simulink model "Three_Stages"  (R2023a)
settings: Solver=FixedStepDiscrete  StartTime=0.0  StopTime=5000  FixedStep=1  RelTol=1e-3
values from neighbouring files (symbols this model uses):
  fw = zeros(16384, 1, 'uint32')    [test.m]
libraries: hdlsllib x27, simulink x27, etargetslib x1
(part 4 of 5)

== system Three_Stages/Subsystem21/Subsystem17 ==
  rst_n : Inport
  stall : Inport  Port=2
  flush : Inport  Port=3
  s_in : Inport  Port=4
  Constant : Constant  Value=0  OutDataTypeStr=boolean
  Constant1 : Constant  Value=0  OutDataTypeStr=uint32
  Resettable Delay : Delay  DelayLength=1  InitialConditionSource=Input port  ExternalReset=Falling
      settings: InputPortMap=u0,r5,p4
  Switch : Switch  Criteria=u2 ~= 0  OutDataTypeStr=boolean  SaturateOnIntegerOverflow=off  InputSameDT=off
  Switch1 : Switch  Criteria=u2 ~= 0  OutDataTypeStr=boolean  SaturateOnIntegerOverflow=off  InputSameDT=off
  s_out : Outport
  wires:
  Constant1/1 -> Switch1/1
  Switch1/1 -> Resettable Delay/1
  Resettable Delay/1 -> s_out/1, Switch/1
  Constant/1 -> Resettable Delay/3
  flush/1 -> Switch1/2
  rst_n/1 -> Resettable Delay/2
  Switch/1 -> Switch1/3
  stall/1 -> Switch/2
  s_in/1 -> Switch/3

== system Three_Stages/Subsystem21/Subsystem18 ==
  rst_n : Inport
  stall : Inport  Port=2
  flush : Inport  Port=3
  valid_in : Inport  Port=4
  Constant : Constant  Value=0  OutDataTypeStr=boolean
  Constant1 : Constant  Value=0  OutDataTypeStr=uint32
  Resettable Delay : Delay  DelayLength=1  InitialConditionSource=Input port  ExternalReset=Falling
      settings: InputPortMap=u0,r5,p4
  Switch : Switch  Criteria=u2 ~= 0  OutDataTypeStr=boolean  SaturateOnIntegerOverflow=off  InputSameDT=off
  Switch1 : Switch  Criteria=u2 ~= 0  OutDataTypeStr=boolean  SaturateOnIntegerOverflow=off  InputSameDT=off
  valid_out : Outport
  wires:
  Constant1/1 -> Switch1/1
  Switch1/1 -> Resettable Delay/1
  Resettable Delay/1 -> valid_out/1, Switch/1
  Constant/1 -> Resettable Delay/3
  flush/1 -> Switch1/2
  rst_n/1 -> Resettable Delay/2
  Switch/1 -> Switch1/3
  stall/1 -> Switch/2
  valid_in/1 -> Switch/3

== system Three_Stages/Subsystem21/Subsystem19 ==
  rst_n : Inport
  stall : Inport  Port=2
  flush : Inport  Port=3
  link_en_in : Inport  Port=4
  Constant : Constant  Value=0  OutDataTypeStr=boolean
  Constant1 : Constant  Value=0  OutDataTypeStr=uint32
  Resettable Delay : Delay  DelayLength=1  InitialConditionSource=Input port  ExternalReset=Falling
      settings: InputPortMap=u0,r5,p4
  Switch : Switch  Criteria=u2 ~= 0  OutDataTypeStr=boolean  SaturateOnIntegerOverflow=off  InputSameDT=off
  Switch1 : Switch  Criteria=u2 ~= 0  OutDataTypeStr=boolean  SaturateOnIntegerOverflow=off  InputSameDT=off
  link_en_out : Outport
  wires:
  Constant1/1 -> Switch1/1
  Switch1/1 -> Resettable Delay/1
  Resettable Delay/1 -> link_en_out/1, Switch/1
  Constant/1 -> Resettable Delay/3
  flush/1 -> Switch1/2
  rst_n/1 -> Resettable Delay/2
  Switch/1 -> Switch1/3
  stall/1 -> Switch/2
  link_en_in/1 -> Switch/3

== system Three_Stages/Subsystem21/Subsystem2 ==
  rst_n : Inport
  stall : Inport  Port=2
  imm32_in : Inport  Port=3
  Constant : Constant  Value=0  OutDataTypeStr=uint32
  Resettable Delay : Delay  DelayLength=1  InitialConditionSource=Input port  ExternalReset=Falling
      settings: InputPortMap=u0,r5,p4
  Switch : Switch  Criteria=u2 ~= 0  SaturateOnIntegerOverflow=off  InputSameDT=off
  imm32_out : Outport
  wires:
  imm32_in/1 -> Switch/3
  Resettable Delay/1 -> imm32_out/1, Switch/1
  Switch/1 -> Resettable Delay/1
  rst_n/1 -> Resettable Delay/2
  Constant/1 -> Resettable Delay/3
  stall/1 -> Switch/2

== system Three_Stages/Subsystem21/Subsystem20 ==
  rst_n : Inport
  stall : Inport  Port=2
  flush : Inport  Port=3
  reg_list_in : Inport  Port=4
  Constant : Constant  Value=0  OutDataTypeStr=uint16
  Constant1 : Constant  Value=0  OutDataTypeStr=uint16
  Resettable Delay : Delay  DelayLength=1  InitialConditionSource=Input port  ExternalReset=Falling
      settings: InputPortMap=u0,r5,p4
  Switch : Switch  Criteria=u2 ~= 0  OutDataTypeStr=uint16  SaturateOnIntegerOverflow=off  InputSameDT=off
  Switch1 : Switch  Criteria=u2 ~= 0  OutDataTypeStr=uint16  SaturateOnIntegerOverflow=off  InputSameDT=off
  reg_list_out : Outport
  wires:
  Constant1/1 -> Switch1/1
  Switch1/1 -> Resettable Delay/1
  Resettable Delay/1 -> reg_list_out/1, Switch/1
  Constant/1 -> Resettable Delay/3
  flush/1 -> Switch1/2
  rst_n/1 -> Resettable Delay/2
  Switch/1 -> Switch1/3
  stall/1 -> Switch/2
  reg_list_in/1 -> Switch/3

== system Three_Stages/Subsystem21/Subsystem21 ==
  rst_n : Inport
  stall : Inport  Port=2
  alu_acc_in : Inport  Port=3
  Constant : Constant  Value=0  OutDataTypeStr=uint32
  Resettable Delay : Delay  DelayLength=1  InitialConditionSource=Input port  ExternalReset=Falling
      settings: InputPortMap=u0,r5,p4
  Switch : Switch  Criteria=u2 ~= 0  SaturateOnIntegerOverflow=off  InputSameDT=off
  alu_acc_out : Outport
  wires:
  alu_acc_in/1 -> Switch/3
  Resettable Delay/1 -> alu_acc_out/1, Switch/1
  Switch/1 -> Resettable Delay/1
  rst_n/1 -> Resettable Delay/2
  Constant/1 -> Resettable Delay/3
  stall/1 -> Switch/2

== system Three_Stages/Subsystem21/Subsystem22 ==
  rst_n : Inport
  stall : Inport  Port=2
  instr_addr_in : Inport  Port=3
  Constant : Constant  Value=0  OutDataTypeStr=uint32
  Resettable Delay : Delay  DelayLength=1  InitialConditionSource=Input port  ExternalReset=Falling
      settings: InputPortMap=u0,r5,p4
  Switch : Switch  Criteria=u2 ~= 0  SaturateOnIntegerOverflow=off  InputSameDT=off
  id_instr_addr_out : Outport
  wires:
  instr_addr_in/1 -> Switch/3
  Resettable Delay/1 -> id_instr_addr_out/1, Switch/1
  Switch/1 -> Resettable Delay/1
  rst_n/1 -> Resettable Delay/2
  Constant/1 -> Resettable Delay/3
  stall/1 -> Switch/2

== system Three_Stages/Subsystem21/Subsystem25 ==
  rst_n : Inport
  stall : Inport  Port=2
  rd_lo_in : Inport  Port=3
  Constant : Constant  Value=0  OutDataTypeStr=uint32
  Resettable Delay : Delay  DelayLength=1  InitialConditionSource=Input port  ExternalReset=Falling
      settings: InputPortMap=u0,r5,p4
  Switch : Switch  Criteria=u2 ~= 0  SaturateOnIntegerOverflow=off  InputSameDT=off
  rd_lo_out : Outport
  wires:
  rd_lo_in/1 -> Switch/3
  Resettable Delay/1 -> rd_lo_out/1, Switch/1
  Switch/1 -> Resettable Delay/1
  rst_n/1 -> Resettable Delay/2
  Constant/1 -> Resettable Delay/3
  stall/1 -> Switch/2

== system Three_Stages/Subsystem21/Subsystem26 ==
  rst_n : Inport
  stall : Inport  Port=2
  rd_hi_in : Inport  Port=3
  Constant : Constant  Value=0  OutDataTypeStr=uint32
  Resettable Delay : Delay  DelayLength=1  InitialConditionSource=Input port  ExternalReset=Falling
      settings: InputPortMap=u0,r5,p4
  Switch : Switch  Criteria=u2 ~= 0  SaturateOnIntegerOverflow=off  InputSameDT=off
  rd_hi_out : Outport
  wires:
  rd_hi_in/1 -> Switch/3
  Resettable Delay/1 -> rd_hi_out/1, Switch/1
  Switch/1 -> Resettable Delay/1
  rst_n/1 -> Resettable Delay/2
  Constant/1 -> Resettable Delay/3
  stall/1 -> Switch/2

== system Three_Stages/Subsystem21/Subsystem27 ==
  rst_n : Inport
  stall : Inport  Port=2
  two_wb_in : Inport  Port=3
  Constant : Constant  Value=0  OutDataTypeStr=uint32
  Resettable Delay : Delay  DelayLength=1  InitialConditionSource=Input port  ExternalReset=Falling
      settings: InputPortMap=u0,r5,p4
  Switch : Switch  Criteria=u2 ~= 0  SaturateOnIntegerOverflow=off  InputSameDT=off
  two_wb_out : Outport
  wires:
  two_wb_in/1 -> Switch/3
  Resettable Delay/1 -> two_wb_out/1, Switch/1
  Switch/1 -> Resettable Delay/1
  rst_n/1 -> Resettable Delay/2
  Constant/1 -> Resettable Delay/3
  stall/1 -> Switch/2

== system Three_Stages/Subsystem21/Subsystem4 ==
  rst_n : Inport
  stall : Inport  Port=2
  rd_in : Inport  Port=3
  Constant : Constant  Value=0  OutDataTypeStr=uint8
  Resettable Delay : Delay  DelayLength=1  InitialConditionSource=Input port  ExternalReset=Falling
      settings: InputPortMap=u0,r5,p4
  Switch : Switch  Criteria=u2 ~= 0  SaturateOnIntegerOverflow=off  InputSameDT=off
  rd_out : Outport
  wires:
  rd_in/1 -> Switch/3
  Resettable Delay/1 -> rd_out/1, Switch/1
  Switch/1 -> Resettable Delay/1
  rst_n/1 -> Resettable Delay/2
  Constant/1 -> Resettable Delay/3
  stall/1 -> Switch/2

== system Three_Stages/Subsystem21/Subsystem5 ==
  rst_n : Inport
  stall : Inport  Port=2
  rn_in : Inport  Port=3
  Constant : Constant  Value=0  OutDataTypeStr=uint8
  Resettable Delay : Delay  DelayLength=1  InitialConditionSource=Input port  ExternalReset=Falling
      settings: InputPortMap=u0,r5,p4
  Switch : Switch  Criteria=u2 ~= 0  SaturateOnIntegerOverflow=off  InputSameDT=off
  rn_out : Outport
  wires:
  rn_in/1 -> Switch/3
  Resettable Delay/1 -> rn_out/1, Switch/1
  Switch/1 -> Resettable Delay/1
  rst_n/1 -> Resettable Delay/2
  Constant/1 -> Resettable Delay/3
  stall/1 -> Switch/2

== system Three_Stages/Subsystem21/Subsystem6 ==
  rst_n : Inport
  stall : Inport  Port=2
  rm_in : Inport  Port=3
  Constant : Constant  Value=0  OutDataTypeStr=uint8
  Resettable Delay : Delay  DelayLength=1  InitialConditionSource=Input port  ExternalReset=Falling
      settings: InputPortMap=u0,r5,p4
  Switch : Switch  Criteria=u2 ~= 0  SaturateOnIntegerOverflow=off  InputSameDT=off
  rm_out : Outport
  wires:
  rm_in/1 -> Switch/3
  Resettable Delay/1 -> rm_out/1, Switch/1
  Switch/1 -> Resettable Delay/1
  rst_n/1 -> Resettable Delay/2
  Constant/1 -> Resettable Delay/3
  stall/1 -> Switch/2

== system Three_Stages/Subsystem21/Subsystem7 ==
  rst_n : Inport
  stall : Inport  Port=2
  WB_addr_in : Inport  Port=3
  Constant : Constant  Value=0  OutDataTypeStr=uint32
  Resettable Delay : Delay  DelayLength=1  InitialConditionSource=Input port  ExternalReset=Falling
      settings: InputPortMap=u0,r5,p4
  Switch : Switch  Criteria=u2 ~= 0  SaturateOnIntegerOverflow=off  InputSameDT=off
  WB_addr_out : Outport
  wires:
  WB_addr_in/1 -> Switch/3
  Resettable Delay/1 -> WB_addr_out/1, Switch/1
  Switch/1 -> Resettable Delay/1
  rst_n/1 -> Resettable Delay/2
  Constant/1 -> Resettable Delay/3
  stall/1 -> Switch/2

== system Three_Stages/Subsystem21/Subsystem8 ==
  rst_n : Inport
  stall : Inport  Port=2
  alu_op_in : Inport  Port=3
  Constant : Constant  Value=12  OutDataTypeStr=uint32
  Resettable Delay : Delay  DelayLength=1  InitialConditionSource=Input port  ExternalReset=Falling
      settings: InputPortMap=u0,r5,p4
  Switch : Switch  Criteria=u2 ~= 0  SaturateOnIntegerOverflow=off  InputSameDT=off
  alu_op_out : Outport
  wires:
  alu_op_in/1 -> Switch/3
  Resettable Delay/1 -> alu_op_out/1, Switch/1
  Switch/1 -> Resettable Delay/1
  rst_n/1 -> Resettable Delay/2
  Constant/1 -> Resettable Delay/3
  stall/1 -> Switch/2

== system Three_Stages/Subsystem21/Subsystem9 ==
  rst_n : Inport
  stall : Inport  Port=2
  alu_src_b_in : Inport  Port=3
  Constant : Constant  Value=0  OutDataTypeStr=boolean
  Resettable Delay : Delay  DelayLength=1  InitialConditionSource=Input port  ExternalReset=Falling
      settings: InputPortMap=u0,r5,p4
  Switch : Switch  Criteria=u2 ~= 0  SaturateOnIntegerOverflow=off  InputSameDT=off
  alu_src_b_out : Outport
  wires:
  alu_src_b_in/1 -> Switch/3
  Resettable Delay/1 -> alu_src_b_out/1, Switch/1
  Switch/1 -> Resettable Delay/1
  rst_n/1 -> Resettable Delay/2
  Constant/1 -> Resettable Delay/3
  stall/1 -> Switch/2

== system Three_Stages/Subsystem3/is_load_op ==
  opcode_out : Inport
  Constant : Constant  Value=15  OutDataTypeStr=uint8
  Constant1 : Constant  Value=49  OutDataTypeStr=uint8
  Constant2 : Constant  Value=58  OutDataTypeStr=uint8
  Constant3 : Constant  Value=77  OutDataTypeStr=uint8
  Constant4 : Constant  Value=80  OutDataTypeStr=uint8
  Constant5 : Constant  Value=81  OutDataTypeStr=uint8
  Constant6 : Constant  Value=103  OutDataTypeStr=uint8
  Logical Operator : Logic  Operator=OR  Inputs=7  AllPortsSameDT=off  OutDataTypeStr=boolean
  Relational Operator{,1..6} (7 alike) : RelationalOperator  Operator===  OutDataTypeStr=boolean  RndMeth=Simplest  InputSameDT=off
  Out1 : Outport
  wires:
  opcode_out/1 -> Relational Operator6/1, Relational Operator5/1, Relational Operator4/1, Relational Operator3/1, Relational Operator2/1, Relational Operator1/1, Relational Operator/1  "op"
  Constant/1 -> Relational Operator/2
  Relational Operator/1 -> Logical Operator/1
  Relational Operator1/1 -> Logical Operator/2
  Relational Operator2/1 -> Logical Operator/3
  Relational Operator3/1 -> Logical Operator/4
  Relational Operator4/1 -> Logical Operator/5
  Relational Operator5/1 -> Logical Operator/6
  Logical Operator/1 -> Out1/1  "ex_is_load"
  Constant1/1 -> Relational Operator1/2
  Constant2/1 -> Relational Operator2/2
  Constant3/1 -> Relational Operator3/2
  Constant4/1 -> Relational Operator4/2
  Constant5/1 -> Relational Operator5/2
  Relational Operator6/1 -> Logical Operator/7
  Constant6/1 -> Relational Operator6/2

== system Three_Stages/Subsystem3/is_multi_load_op ==
  opcode_out : Inport
  Constant : Constant  Value=78  OutDataTypeStr=uint8
  Constant1 : Constant  Value=69  OutDataTypeStr=uint8
  Constant2 : Constant  Value=87  OutDataTypeStr=uint8
  Constant3 : Constant  Value=39  OutDataTypeStr=uint8
  Constant4 : Constant  Value=40  OutDataTypeStr=uint8
  Constant5 : Constant  Value=41  OutDataTypeStr=uint8
  Constant6 : Constant  Value=90  OutDataTypeStr=uint8
  Logical Operator : Logic  Operator=OR  Inputs=7  AllPortsSameDT=off  OutDataTypeStr=boolean
  Relational Operator{,1..6} (7 alike) : RelationalOperator  Operator===  OutDataTypeStr=boolean  RndMeth=Simplest  InputSameDT=off
  Out1 : Outport
  wires:
  opcode_out/1 -> Relational Operator6/1, Relational Operator5/1, Relational Operator4/1, Relational Operator3/1, Relational Operator2/1, Relational Operator1/1, Relational Operator/1  "op"
  Constant/1 -> Relational Operator/2
  Relational Operator/1 -> Logical Operator/1
  Relational Operator1/1 -> Logical Operator/2
  Relational Operator2/1 -> Logical Operator/3
  Relational Operator3/1 -> Logical Operator/4
  Relational Operator4/1 -> Logical Operator/5
  Relational Operator5/1 -> Logical Operator/6
  Logical Operator/1 -> Out1/1  "ex_is_multi_ld"
  Constant1/1 -> Relational Operator1/2
  Constant2/1 -> Relational Operator2/2
  Constant3/1 -> Relational Operator3/2
  Constant4/1 -> Relational Operator4/2
  Constant5/1 -> Relational Operator5/2
  Relational Operator6/1 -> Logical Operator/7
  Constant6/1 -> Relational Operator6/2

== system Three_Stages/Subsystem3/is_multi_store_op ==
  opcode_out : Inport
  Constant : Constant  Value=79  OutDataTypeStr=uint8
  Constant1 : Constant  Value=68  OutDataTypeStr=uint8
  Constant2 : Constant  Value=37  OutDataTypeStr=uint8
  Constant3 : Constant  Value=38  OutDataTypeStr=uint8
  Constant4 : Constant  Value=113  OutDataTypeStr=uint8
  Logical Operator : Logic  Operator=OR  Inputs=5  AllPortsSameDT=off  OutDataTypeStr=boolean
  Relational Operator{,1..4} (5 alike) : RelationalOperator  Operator===  OutDataTypeStr=boolean  RndMeth=Simplest  InputSameDT=off
  Out1 : Outport
  wires:
  opcode_out/1 -> Relational Operator4/1, Relational Operator3/1, Relational Operator2/1, Relational Operator1/1, Relational Operator/1  "op"
  Constant/1 -> Relational Operator/2
  Relational Operator/1 -> Logical Operator/1
  Relational Operator1/1 -> Logical Operator/2
  Relational Operator2/1 -> Logical Operator/3
  Relational Operator3/1 -> Logical Operator/4
  Logical Operator/1 -> Out1/1  "ex_is_multi_st"
  Constant1/1 -> Relational Operator1/2
  Constant2/1 -> Relational Operator2/2
  Constant3/1 -> Relational Operator3/2
  Relational Operator4/1 -> Logical Operator/5
  Constant4/1 -> Relational Operator4/2

== system Three_Stages/Subsystem3/is_store_op ==
  opcode_out : Inport
  Constant : Constant  Value=17  OutDataTypeStr=uint8
  Constant1 : Constant  Value=22  OutDataTypeStr=uint8
  Constant2 : Constant  Value=50  OutDataTypeStr=uint8
  Constant3 : Constant  Value=56  OutDataTypeStr=uint8
  Constant4 : Constant  Value=63  OutDataTypeStr=uint8
  Constant5 : Constant  Value=73  OutDataTypeStr=uint8
  Constant6 : Constant  Value=74  OutDataTypeStr=uint8
  Constant7 : Constant  Value=75  OutDataTypeStr=uint8
  Constant8 : Constant  Value=76  OutDataTypeStr=uint8
  Logical Operator : Logic  Operator=OR  Inputs=9  AllPortsSameDT=off  OutDataTypeStr=boolean
  Relational Operator{,1..8} (9 alike) : RelationalOperator  Operator===  OutDataTypeStr=boolean  RndMeth=Simplest  InputSameDT=off
  Out1 : Outport
  wires:
  opcode_out/1 -> Relational Operator8/1, Relational Operator7/1, Relational Operator6/1, Relational Operator5/1, Relational Operator4/1, Relational Operator3/1, Relational Operator2/1, Relational Operator1/1, Relational Operator/1  "op"
  Constant/1 -> Relational Operator/2
  Relational Operator/1 -> Logical Operator/1
  Relational Operator1/1 -> Logical Operator/2
  Relational Operator2/1 -> Logical Operator/3
  Relational Operator3/1 -> Logical Operator/4
  Relational Operator4/1 -> Logical Operator/5
  Relational Operator5/1 -> Logical Operator/6
  Logical Operator/1 -> Out1/1  "ex_is_store"
  Constant1/1 -> Relational Operator1/2
  Constant2/1 -> Relational Operator2/2
  Constant3/1 -> Relational Operator3/2
  Constant4/1 -> Relational Operator4/2
  Constant5/1 -> Relational Operator5/2
  Relational Operator6/1 -> Logical Operator/7
  Relational Operator7/1 -> Logical Operator/8
  Relational Operator8/1 -> Logical Operator/9
  Constant6/1 -> Relational Operator6/2
  Constant7/1 -> Relational Operator7/2
  Constant8/1 -> Relational Operator8/2

== system Three_Stages/Subsystem4/Subsystem3 ==
  In1 : Inport
  In2 : Inport  Port=2
  Constant : Constant  Value=0  OutDataTypeStr=boolean
  Resettable Delay : Delay  DelayLength=1  InitialConditionSource=Input port  ExternalReset=Falling
      settings: InputPortMap=u0,r5,p4
  Out1 : Outport
  wires:
  Constant/1 -> Resettable Delay/3
  In1/1 -> Resettable Delay/1  "flush"
  In2/1 -> Resettable Delay/2  "rst_n"
  Resettable Delay/1 -> Out1/1  "flush_apsr_d"

== system Three_Stages/MR/Subsystem6/Subsystem ==
  In1 : Inport
  In2 : Inport  Port=2
  In3 : Inport  Port=3
  In4 : Inport  Port=4
  In5 : Inport  Port=5
  In6 : Inport  Port=6
  Constant : Constant  OutDataTypeStr=uint8
  Constant1 : Constant  Value=0  OutDataTypeStr=uint8
  Constant2 : Constant  Value=2  OutDataTypeStr=uint8
  Constant3 : Constant  Value=3  OutDataTypeStr=uint8
  Constant4 : Constant  Value=4  OutDataTypeStr=uint8
  Constant5 : Constant  Value=5  OutDataTypeStr=uint8
  Constant6 : Constant  Value=6  OutDataTypeStr=uint8
  Switch{,1..5} (6 alike) : Switch  Criteria=u2 ~= 0  SaturateOnIntegerOverflow=off  InputSameDT=off
  Out1 : Outport
  wires:
  Constant/1 -> Switch5/1
  Switch5/1 -> Switch4/3
  Switch4/1 -> Switch3/3
  Switch3/1 -> Switch2/3
  Switch2/1 -> Switch1/3
  Switch1/1 -> Switch/3
  Constant1/1 -> Switch5/3
  In1/1 -> Switch5/2  "eq_ldm_w"
  In2/1 -> Switch4/2  "eq_ldm_w_nwb"
  Constant2/1 -> Switch4/1
  Constant3/1 -> Switch3/1
  Constant6/1 -> Switch/1
  Constant5/1 -> Switch1/1
  Constant4/1 -> Switch2/1
  In3/1 -> Switch3/2  "eq_pop"
  In4/1 -> Switch2/2  "eq_stm"
  In5/1 -> Switch1/2  "eq_push"
  In6/1 -> Switch/2  "eq_ldrd"
  Switch/1 -> Out1/1  "mr_op_decoded"

== matlab function Three_Stages/memory/MATLAB Function1 ==
  data: rst_n input; read_data output; write_en input; write_addr input; write_data input; read_en input; read_addr input; instr_addr input; instr_data output; fw_init input
function [read_data, instr_data] = memory(rst_n, ...
    write_en, write_addr, write_data, ...
    read_en, read_addr, instr_addr, fw_init)
% =========================================================
% Memory Module: Flash (16384 words) + SRAM (5120 words)
% 同步写、组合读
% fw_init: 固件镜像（16384x1 uint32），首拍拷贝进 Flash
% 注意: rst_n 端口仅为接口对齐，存储内容不复位
% =========================================================

    %#ok<*INUSD>  % rst_n 故意不使用

    % ---------- 常量 ----------
    FLASH_DEPTH = uint32(16384);
    SRAM_DEPTH  = uint32(5120);
    FLASH_BASE  = uint32(134217728);    % 0x08000000
    SRAM_BASE   = uint32(536870912);    % 0x20000000
    ALIAS_BASE  = uint32(hex2dec('22000000'));   % 0x22000000 位带别名区
    ALIAS_DEPTH = uint32(1024);                  % 别名区独立 4KB，与 SRAM 互不干扰
    BUBBLE_INSTR = uint32(48896);

    % ---------- persistent 存储阵列 ----------
    persistent flash_reg sram_reg alias_reg
    if isempty(flash_reg)
        flash_reg = fw_init;
        sram_reg  = zeros(double(SRAM_DEPTH), 'uint32');
        alias_reg = zeros(double(ALIAS_DEPTH), 'uint32');
    end

    % =========================================================
    % 同步写
    % =========================================================
    if write_en
        if (write_addr >= FLASH_BASE) && ...
           (write_addr < FLASH_BASE + FLASH_DEPTH * uint32(4))
            widx = double(bitshift(write_addr - FLASH_BASE, -2));
            if (widx >= 0) && (widx < double(FLASH_DEPTH))
                flash_reg(widx + 1) = uint32(write_data);
            end
        elseif (write_addr >= SRAM_BASE) && ...
               (write_addr < SRAM_BASE + SRAM_DEPTH * uint32(4))
            widx = double(bitshift(write_addr - SRAM_BASE, -2));
            if (widx >= 0) && (widx < double(SRAM_DEPTH))
                sram_reg(widx + 1) = uint32(write_data);
            end
        elseif (write_addr >= ALIAS_BASE) && ...
               (write_addr < ALIAS_BASE + ALIAS_DEPTH * uint32(4))
            widx = double(bitshift(write_addr - ALIAS_BASE, -2));
            if (widx >= 0) && (widx < double(ALIAS_DEPTH))
                alias_reg(widx + 1) = uint32(write_data);
            end
        end
    end

    % =========================================================
    % 组合读（数据端口）
    % =========================================================
    read_data = uint32(0);
    if read_en
        if (read_addr >= FLASH_BASE) && ...
           (read_addr < FLASH_BASE + FLASH_DEPTH * uint32(4))
            ridx = double(bitshift(read_addr - FLASH_BASE, -2));
            if (ridx >= 0) && (ridx < double(FLASH_DEPTH))
                read_data = flash_reg(ridx + 1);
            end
        elseif (read_addr >= SRAM_BASE) && ...
               (read_addr < SRAM_BASE + SRAM_DEPTH * uint32(4))
            ridx = double(bitshift(read_addr - SRAM_BASE, -2));
            if (ridx >= 0) && (ridx < double(SRAM_DEPTH))
                read_data = sram_reg(ridx + 1);
            end
        elseif (read_addr >= ALIAS_BASE) && ...
               (read_addr < ALIAS_BASE + ALIAS_DEPTH * uint32(4))
            ridx = double(bitshift(read_addr - ALIAS_BASE, -2));
            if (ridx >= 0) && (ridx < double(ALIAS_DEPTH))
                read_data = alias_reg(ridx + 1);
            end
        end
    end

    % =========================================================
    % 组合读（IF 端口）：只读 Flash，越界返回 BKPT
    % =========================================================
    instr_data = BUBBLE_INSTR;
    if (instr_addr >= FLASH_BASE) && ...
       (instr_addr < FLASH_BASE + FLASH_DEPTH * uint32(4))
        iidx = double(bitshift(instr_addr - FLASH_BASE, -2));
        if (iidx >= 0) && (iidx < double(FLASH_DEPTH))
            instr_data = flash_reg(iidx + 1);
        end
    end
end

== matlab function Three_Stages/Prefetch_Unit/Subsystem/MATLAB Function ==
  data: fifo_mem input; next_fifo_mem output; wr_ptr input; rd_ptr input; count input; fetch_pc input; instr input; instr_width input; pop_valid input; instr_data input; flush input; flush_target input; stall input; next_wr_ptr output; next_rd_ptr output; next_count output; next_fetch_pc output; next_instr output; next_instr_width output; next_pop_valid output
function [next_fifo_mem, next_wr_ptr, next_rd_ptr, next_count, ...
          next_fetch_pc, next_instr, next_instr_width, next_pop_valid] = ...
    prefetch_next(...
        fifo_mem, wr_ptr, rd_ptr, count, ...
        fetch_pc, instr, instr_width, pop_valid, ...
        instr_data, flush, flush_target, stall)
%#codegen
% =========================================================
% Prefetch_Unit 的 next-state 组合逻辑（修复版）
%   - FIFO 颗粒度：半字（16 位）
%   - 每拍最多填 2 个半字（字对齐时填 2，非对齐时填 1）
%   - 消费：16 位 pop 1 个；32 位 pop 2 个
%   - stall 时整体保持
%   - flush 时只清空 FIFO 并把 fetch_pc 跳到 flush_target，
%     【不在 flush 拍填充】，避免把 delay unit 之后的旧数据填入。
%
% ★ 修复说明（2026-10-16）★
%   原版缺陷：fetch_pc 的前进（+4 / +2）写在 fill 数据计算块里，
%   【没有受 can_fill 控制】。当 FIFO 已满(count==8)且队首是 16 位
%   指令时：pop 1 个半字 → count_after_pop=7 → 7+2>8 → can_fill=false
%   → 本拍不填充，但 fetch_pc 仍然 +4！于是 instr_data 对应的那个字
%   被永久跳过，FIFO 半字流从此错位 2 个半字，下游取出错误指令
%   （例如 0x8000282 处的 f4bfaff7 被取成 f4bfbf28）。
%   修复：fetch_pc 只在真正填充（can_fill 为真）时才前进，否则保持。
% =========================================================

    FIFO_DEPTH = 6;

    % ---------- 默认值（保持） ----------
    next_fifo_mem    = fifo_mem;
    next_wr_ptr      = wr_ptr;
    next_rd_ptr      = rd_ptr;
    next_count       = count;
    next_fetch_pc    = fetch_pc;   % ★ 默认保持；只有 can_fill 时才前进
    next_instr       = instr;
    next_instr_width = instr_width;
    next_pop_valid   = pop_valid;

    % ============ flush：只清空 + 跳 fetch_pc，不填充 ============
    if flush
        next_fifo_mem(:) = uint16(0);
        next_wr_ptr      = uint8(0);
        next_rd_ptr      = uint8(0);
        next_count       = uint8(0);
        next_fetch_pc    = uint32(flush_target);
        next_instr       = uint32(0);
        next_instr_width = false;
        next_pop_valid   = false;
        return;
    end

    % ============ stall（完全保持）============
    if stall
        return;
    end

    % ============ 指针 ============
    wr_p1 = uint8(mod(double(wr_ptr) + 1, FIFO_DEPTH));
    wr_p2 = uint8(mod(double(wr_ptr) + 2, FIFO_DEPTH));
    rd_p1 = uint8(mod(double(rd_ptr) + 1, FIFO_DEPTH));

    % ============ head halfword 分析 ============
    head_h0 = fifo_mem(double(rd_ptr) + 1);
    head_h1 = fifo_mem(double(rd_p1) + 1);

    % Thumb-2 32 位指令前导半字高 5 位 ∈ {11101, 11110, 11111}
    top5 = bitshift(head_h0, -11);
    head_is_32 = (top5 == uint16(29)) || ...
                 (top5 == uint16(30)) || ...
                 (top5 == uint16(31));

    % ============ pop 判断 ============
    can_pop_16 = (count >= uint8(1)) && ~head_is_32;
    can_pop_32 = (count >= uint8(2)) &&  head_is_32;
    can_pop    = can_pop_16 || can_pop_32;
    pop_2      = can_pop_32;

    if ~can_pop
        pop_amt = uint8(0);
    elseif pop_2
        pop_amt = uint8(2);
    else
        pop_amt = uint8(1);
    end

    % ============ fill 数据准备（只算数据，不动 fetch_pc）============
    if bitand(bitshift(fetch_pc, -1), uint32(1)) == 0
        % 字对齐：一次填 2 个半字
        fill_data_lo  = uint16(bitand(instr_data, uint32(65535)));
        fill_data_hi  = uint16(bitshift(instr_data, -16));
        fill_count    = uint8(2);
    else
        % 半字对齐：只填高半字，填 1 个
        fill_data_lo  = uint16(bitshift(instr_data, -16));
        fill_data_hi  = uint16(0);
        fill_count    = uint8(1);
    end

    count_after_pop = double(count) - double(pop_amt);
    can_fill        = (count_after_pop + double(fill_count) <= FIFO_DEPTH);

    % ============ pop 输出 ============
    if can_pop
        if pop_2
            next_instr       = bitor(bitshift(uint32(head_h0), 16), uint32(head_h1));
            next_instr_width = true;
            next_rd_ptr      = uint8(mod(double(rd_ptr) + 2, FIFO_DEPTH));
        else
            next_instr       = uint32(head_h0);
            next_instr_width = false;
            next_rd_ptr      = rd_p1;
        end
        next_pop_valid = true;
    else
        next_pop_valid = false;
    end

    % ============ fill 输出 + fetch_pc 前进（必须同生共死）============
    if can_fill
        next_fifo_mem(double(wr_ptr) + 1) = fill_data_lo;
        if fill_count == 2
            next_fifo_mem(double(wr_p1) + 1) = fill_data_hi;
            next_wr_ptr   = wr_p2;
            next_fetch_pc = fetch_pc + uint32(4);   % ★ 只在填充时前进
        else
            next_wr_ptr   = wr_p1;
            next_fetch_pc = fetch_pc + uint32(2);   % ★ 只在填充时前进
        end
        next_count = uint8(count_after_pop + double(fill_count));
    else
        % ★ 不填充：wr_ptr 与 fetch_pc 都必须原地保持，
        %   否则本拍 instr_data 对应的字会被永久跳过
        next_wr_ptr   = wr_ptr;
        next_fetch_pc = fetch_pc;
        next_count    = uint8(count_after_pop);
    end
end

== matlab function Three_Stages/Branch_Unit/Subsystem/MATLAB Function ==
  data: id_instr input; cond_pass output; id_instr_width input; id_pc input; id_valid input; id_opcode input; id_cond input; id_rm_data input; fwd_z input; fwd_n input; fwd_c input; fwd_v input; opcode_sel output; target_b output; target_bw output; target_bcond output; target_bl output; target_bx output; target_cbz output; cbz_taken output; cbnz_taken output
function [cond_pass, opcode_sel, target_b, target_bw, target_bcond, ...
          target_bl, target_bx, target_cbz, cbz_taken, cbnz_taken] = ...
    branch_comb(id_instr, id_instr_width, id_pc, id_valid, ...
                id_opcode, id_cond, id_rm_data, ...
                fwd_z, fwd_n, fwd_c, fwd_v)
% =========================================================
% Branch_Unit 组合逻辑（不含最终 MUX）
% ★ 所有 PC + offset 的加法都用有符号 int32 做，避免 Saturate
% =========================================================

    % ---------- 默认输出 ----------
    cond_pass  = false;
    opcode_sel = uint8(14);
    target_b      = uint32(0);
    target_bw     = uint32(0);
    target_bcond  = uint32(0);
    target_bl     = uint32(0);
    target_bx     = uint32(0);
    target_cbz    = uint32(0);
    cbz_taken  = false;
    cbnz_taken = false;

    % ---------- opcode 常量 ----------
    OP_B        = uint8(23);
    OP_B_W      = uint8(52);
    OP_BEQ      = uint8(24);
    OP_BNE      = uint8(27);
    OP_BLT      = uint8(59);
    OP_BLE      = uint8(65);
    OP_BHI      = uint8(82);
    OP_B_COND_W = uint8(71);
    OP_BL       = uint8(34);
    OP_BX       = uint8(51);
    OP_CBZ      = uint8(25);
    OP_CBNZ     = uint8(66);
    OP_BGE      = uint8(89);

    % =========================================================
    % [1] cond_pass
    % =========================================================
    switch id_cond
        case 0,  cond_pass = fwd_z;
        case 1,  cond_pass = ~fwd_z;
        case 2,  cond_pass = fwd_c;
        case 3,  cond_pass = ~fwd_c;
        case 4,  cond_pass = fwd_n;
        case 5,  cond_pass = ~fwd_n;
        case 6,  cond_pass = fwd_v;
        case 7,  cond_pass = ~fwd_v;
        case 8,  cond_pass = fwd_c && ~fwd_z;
        case 9,  cond_pass = ~fwd_c || fwd_z;
        case 10, cond_pass = (fwd_n == fwd_v);
        case 11, cond_pass = (fwd_n ~= fwd_v);
        case 12, cond_pass = ~fwd_z && (fwd_n == fwd_v);
        case 13, cond_pass = fwd_z || (fwd_n ~= fwd_v);
        case 14, cond_pass = true;
        otherwise, cond_pass = false;
    end

    % =========================================================
    % [2] PC 相关的有符号基准
    % =========================================================
    pc_signed = int32(id_pc) + int32(4);

    % =========================================================
    % [3] 5 个偏移量
    % =========================================================
    instr = uint32(id_instr);

    % ---- b16_offset ----
    imm11 = int32(bitand(instr, uint32(hex2dec('7FF'))));
    if bitget(instr, 11)                 % MATLAB 1-based，对应硬件 bit 10
        imm11 = imm11 - int32(hex2dec('800'));
    end
    b16_raw = bitshift(imm11, 1);
    target_b = uint32(pc_signed + b16_raw);

    % ---- bcond16_offset ----
    bcond16_raw = int32(bitshift(bitand(instr, uint32(255)), 1));
    if bitget(instr, 8)                  % MATLAB 1-based，对应硬件 bit 7
        bcond16_raw = bcond16_raw - int32(hex2dec('200'));
    end
    target_bcond = uint32(pc_signed + bcond16_raw);

    % ---- cbz_offset ----
    cbz_raw = uint32(bitor(bitshift(uint32(bitget(instr, 10)), 6), ...
                           bitshift(bitand(bitshift(instr, -3), uint32(31)), 1)));
    target_cbz = uint32(pc_signed + int32(cbz_raw));

    % ---- b32_offset_ext（B<c>.W）----
    % ★ 你原来的代码完全正确！MATLAB bitget 从1开始，27就是硬件的bit26
    b32_S = uint32(bitget(instr, 27));   % 硬件 bit 26 (S)
    J2    = uint32(bitget(instr, 12));   % 硬件 bit 11 (J2)
    J1    = uint32(bitget(instr, 14));   % 硬件 bit 13 (J1)
    imm6  = bitand(bitshift(instr, -16), uint32(63));
    imm11_b32 = bitand(instr, uint32(hex2dec('7FF'))); % 改名防止覆盖前面的 imm11

    b32_raw_unsigned = bitor(bitshift(b32_S, 20), ...
                       bitor(bitshift(J2, 19), ...
                       bitor(bitshift(J1, 18), ...
                       bitor(bitshift(imm6, 12), ...
                       bitor(bitshift(imm11_b32, 1), 0)))));

    b32_signed = int32(b32_raw_unsigned);
    if bitget(b32_raw_unsigned, 21)      % MATLAB 1-based，对应硬件 bit 20
        b32_signed = b32_signed - int32(hex2dec('200000'));
    end
    target_bw = uint32(pc_signed + b32_signed);

    % ---- bl_offset_ext（BL）----
    S_bit = uint32(bitget(instr, 27));   % 硬件 bit 26
    J1_bl = uint32(bitget(instr, 14));   % 硬件 bit 13
    J2_bl = uint32(bitget(instr, 12));   % 硬件 bit 11
    I1    = uint32(~(J1_bl ~= S_bit));
    I2    = uint32(~(J2_bl ~= S_bit));
    imm10 = bitand(bitshift(instr, -16), uint32(1023));

    bl_raw_unsigned = bitor(bitshift(S_bit, 24), ...
                      bitor(bitshift(I1, 23), ...
                      bitor(bitshift(I2, 22), ...
                      bitor(bitshift(imm10, 12), ...
                      bitor(bitshift(imm11_b32, 1), 0)))));

    bl_signed = int32(bl_raw_unsigned);
    if bitget(bl_raw_unsigned, 25)       % MATLAB 1-based，对应硬件 bit 24
        bl_signed = bl_signed - int32(hex2dec('2000000'));
    end
    target_bl = uint32(pc_signed + bl_signed);

    % ---- BX target ----
    target_bx = bitand(id_rm_data, uint32(hex2dec('FFFFFFFE')));

    % =========================================================
    % [4] cbz_taken / cbnz_taken
    % =========================================================
    cbz_taken  = (id_rm_data == uint32(0));
    cbnz_taken = (id_rm_data ~= uint32(0));

    % =========================================================
    % [5] opcode_sel 译码
    % =========================================================
    if ~id_valid
        opcode_sel = uint8(14);
        return;
    end

    if id_opcode == OP_B
        opcode_sel = uint8(0);
    elseif id_opcode == OP_B_W
        opcode_sel = uint8(1);
    elseif id_opcode == OP_BEQ
        opcode_sel = uint8(2);
    elseif id_opcode == OP_BNE
        opcode_sel = uint8(3);
    elseif id_opcode == OP_BLT
        opcode_sel = uint8(4);
    elseif id_opcode == OP_BLE
        opcode_sel = uint8(5);
    elseif id_opcode == OP_BHI
        opcode_sel = uint8(6);
    elseif id_opcode == OP_BGE
        opcode_sel = uint8(7);
    elseif id_opcode == OP_B_COND_W
        if id_instr_width == 0
            opcode_sel = uint8(8);
        else
            opcode_sel = uint8(9);
        end
    elseif id_opcode == OP_BL
        opcode_sel = uint8(10);
    elseif id_opcode == OP_BX
        opcode_sel = uint8(11);
    elseif id_opcode == OP_CBZ
        opcode_sel = uint8(12);
    elseif id_opcode == OP_CBNZ
        opcode_sel = uint8(13);
    else
        opcode_sel = uint8(14);
    end
end

== matlab function Three_Stages/Subsystem2/Subsystem1/MATLAB Function1 ==
  data: instr input; instr_width input; instr_valid input; opcode output; it_cond_reg input; it_active_reg input; s output; cond output; valid output; rd output; rn output; rm output; ra output; ra_valid output; rd_lo output; rd_hi output; two_wb output; imm24 output; imm32 output; read_addr_1 output; read_en_1 output; read_addr_2 output; read_en_2 output; write_en output; alu_op output; alu_src_b output; alu_use_carry output; alu_shamt output; alu_shift_type output; reg_list output
function [opcode, s, cond, valid, rd, rn, rm, ra, ra_valid, ...
          rd_lo, rd_hi, two_wb, imm24, imm32, ...
          read_addr_1, read_en_1, read_addr_2, read_en_2, ...
          write_en, alu_op, alu_src_b, alu_use_carry, alu_shamt, ...
          alu_shift_type, reg_list] = ...
    ID_Comb(instr, instr_width, instr_valid, ...
            it_cond_reg, it_active_reg)
% =========================================================
% ID 阶段纯组合译码（不含 IT 状态机，无 persistent）
% =========================================================
%#codegen

    % ---------- 输入类型断言 ----------
    assert(isa(instr, 'uint32'));
    assert(isa(instr_width, 'logical'));
    assert(isa(instr_valid, 'logical'));
    assert(isa(it_cond_reg, 'uint8'));
    assert(isa(it_active_reg, 'logical'));

    % ---------- 常量 ----------
    OP_INV   = uint8(127);
    ALU_PASS = uint8(12);
    SH_LSL   = uint8(0);
    OP_IT    = uint8(67);

    % ---------- 默认输出 ----------
    opcode = OP_INV;
    s = false; cond = uint8(14); valid = true;
    rd = uint8(0); rn = uint8(0); rm = uint8(0);
    ra        = uint8(0);
    ra_valid  = false;
    rd_lo     = uint8(0);
    rd_hi     = uint8(0);
    two_wb    = false;   % ★ 默认不双写
    imm24 = uint32(0); imm32 = uint32(0);
    read_addr_1 = uint8(0); read_en_1 = false;
    read_addr_2 = uint8(0); read_en_2 = false;
    alu_op = ALU_PASS; alu_src_b = false; alu_use_carry = false;
    alu_shamt = uint8(0); alu_shift_type = SH_LSL;
    reg_list = uint16(0);
    write_en = false;

    % ---------- 组合译码 ----------
    if instr_valid
        if instr_width == 0
            [opcode, s, cond, valid, rd, rn, rm, ra, ra_valid, ...
          rd_lo, rd_hi, two_wb, imm24, imm32, ...
             read_addr_1, read_en_1, read_addr_2, read_en_2, ...
             alu_op, alu_src_b, alu_use_carry, alu_shamt, ...
             alu_shift_type, reg_list] = decode_16bit(instr);
        else
            [opcode, s, cond, valid, rd, rn, rm, ra, ra_valid, ...
          rd_lo, rd_hi, two_wb, imm24, imm32, ...
             read_addr_1, read_en_1, read_addr_2, read_en_2, ...
             alu_op, alu_src_b, alu_use_carry, alu_shamt, ...
             alu_shift_type, reg_list] = decode_32bit(instr);
        end
    else
        valid = false;
        opcode = OP_INV;
    end

    % ---------- IT 条件覆盖（用 it_* 输入，不更新状态）----------
    if it_active_reg && opcode ~= OP_IT && opcode ~= OP_INV
        cond = it_cond_reg;
    end
    if opcode == OP_IT
        cond = uint8(bitand(bitshift(instr, -4), uint32(15)));
    end

    % ---------- write_en 判定 ----------
    if valid
        write_opcodes = uint8([0 1 2 3 4 5 6 7 8 9 10 18 19 20 32 ...
                               15 49 58 77 80 81 16 30 21 29 55 ...
                               53 28 42 31 45 54 46 47 70 88 83 72 ...
                               43 60 44 84 86 61 34 62 103 105 109 91 92 107 110 93 94 95]);   % ★ 加 34 (BL)
        if any(opcode == write_opcodes)
            write_en = true;
        end
    end
end

== matlab function Three_Stages/Subsystem2/Subsystem/MATLAB Function2 ==
  data: rst_n input; stall input; instr input; instr_valid input; opcode input; it_cond_next output; it_cond_reg input; it_count_reg input; it_active_reg input; it_count_next output; it_active_next output
function [it_cond_next, it_count_next, it_active_next] = ...
    IT_Next(rst_n, stall, instr, instr_valid, opcode, ...
            it_cond_reg, it_count_reg, it_active_reg)
% =========================================================
% IT 状态机的 next-state 计算（纯组合，无 persistent）
% =========================================================
%#codegen

    % ---------- 类型断言 ----------
    assert(isa(rst_n, 'logical'));
    assert(isa(stall, 'logical'));
    assert(isa(instr, 'uint32'));
    assert(isa(instr_valid, 'logical'));
    assert(isa(opcode, 'uint8'));
    assert(isa(it_cond_reg, 'uint8'));
    assert(isa(it_count_reg, 'uint8'));
    assert(isa(it_active_reg, 'logical'));

    % ---------- 常量 ----------
    OP_IT = uint8(67);

    % ---------- 默认：保持 ----------
    it_cond_next   = it_cond_reg;
    it_count_next  = it_count_reg;
    it_active_next = it_active_reg;

    % ---------- 优先级逻辑 ----------
    if ~rst_n
        % 复位
        it_cond_next   = uint8(14);   % AL
        it_count_next  = uint8(0);
        it_active_next = false;
    elseif ~stall && instr_valid
        if opcode == OP_IT
            % 进入 IT：加载条件码和计数
            it_cond_next   = uint8(bitand(bitshift(instr, -4), uint32(15)));
            it_count_next  = it_count_of_mask(bitand(instr, uint32(15)));
            it_active_next = true;
        elseif it_active_reg
            % 退出或递减
            if it_count_reg <= 1
                it_active_next = false;
                it_count_next  = uint8(0);
            else
                it_count_next  = it_count_reg - uint8(1);
            end
        end
    end
end

== matlab function Three_Stages/MR/MATLAB Function1 ==
  data: state input; mem_re output; pending input; cur_reg input; processed input; total input; addr input; base_reg_r input; base_val input; wb_r input; is_load_r input; is_push_r input; ldrd_rt input; ldrd_rt2 input; mem_rdata input; rf_rd_data input; mem_we output; mem_addr output; mem_wdata output; rf_we output; rf_addr output; rf_wdata output; rf_rd_addr output; rf_rd_en output; load_pc_en output; load_pc_val output; busy output
function [mem_re, mem_we, mem_addr, mem_wdata, ...
          rf_we, rf_addr, rf_wdata, rf_rd_addr, rf_rd_en, ...
          load_pc_en, load_pc_val, busy] = mr_output_decode( ...
    state, pending, cur_reg, processed, total, addr, base_reg_r, base_val, ...
    wb_r, is_load_r, is_push_r, ldrd_rt, ldrd_rt2, ...
    mem_rdata, rf_rd_data)
%#codegen
% =========================================================
% MR Moore 输出译码：只依赖 state 和状态变量
% 修复点：
%   1. 默认 mem_addr 改为 addr，避免状态切换瞬间输出 0
%   2. S_LOAD_CAP 不再发 mem_re，避免重复读
%   3. 删除 S_PC 状态，合并至 S_LOAD_CAP
%   4. 统一 LDRD 读写时序
% =========================================================

% ---------- 状态编码 ----------
S_IDLE       = uint8(0);
S_SCAN       = uint8(1);
S_LOAD_REQ   = uint8(2);
S_LOAD_CAP   = uint8(3);
S_STORE_REQ  = uint8(5);
S_STORE_CAP  = uint8(6);
S_STOREW     = uint8(7);
S_BASE       = uint8(8);
S_LDRD_R1    = uint8(9);
S_LDRD_WB1   = uint8(10);
S_LDRD_R2    = uint8(11);
S_LDRD_WB2   = uint8(12);

% ---------- 默认输出（显式类型） ----------
mem_re      = false;
mem_we      = false;
% ★★★ 关键修改：默认地址设为 addr，保证在 S_SCAN 阶段就提前输出正确地址
mem_addr    = uint32(addr); 
mem_wdata   = uint32(0);
rf_we       = false;
rf_addr     = uint8(0);
rf_wdata    = uint32(0);
rf_rd_addr  = uint8(0);
rf_rd_en    = false;
load_pc_en  = false;
load_pc_val = uint32(0);
busy        = (state ~= S_IDLE);

persistent rdata_cap;
if isempty(rdata_cap), rdata_cap = uint32(0); end

% ---------- 各状态输出 ----------
switch state

    % ---- LOAD 链 ----
    case S_LOAD_REQ
        mem_re   = true;
        mem_addr = uint32(addr);

    case S_LOAD_CAP
        % 捕获数据，不再拉高 mem_re
        mem_addr = uint32(addr);
        if cur_reg == uint8(15)
            load_pc_en  = true;
            load_pc_val = uint32(mem_rdata); 
        else
            rf_we    = true;
            rf_addr  = uint8(cur_reg);
            rf_wdata = uint32(mem_rdata);
        end

    % ---- STORE 链 ----
    case S_STORE_REQ
        rf_rd_addr = uint8(cur_reg);
        rf_rd_en   = true;
        % mem_addr 已由默认值接管，无需显式赋值

    case S_STORE_CAP
        % 保持读使能，等待 rf_rd_data 稳定
        rf_rd_addr = uint8(cur_reg);
        rf_rd_en   = true;
        % mem_addr 已由默认值接管

    case S_STOREW
        % 真正写入内存
        rf_rd_addr = uint8(cur_reg);
        rf_rd_en   = true;
        mem_wdata  = uint32(rf_rd_data);
        mem_addr   = uint32(addr);
        mem_we     = true;

    % ---- 基址写回 ----
    case S_BASE
        rf_we   = logical(wb_r) && (base_reg_r ~= uint8(15));
        rf_addr = uint8(base_reg_r);
        if is_push_r
            rf_wdata = uint32(base_val) - uint32(total) * uint32(4);
        else
            rf_wdata = uint32(base_val) + uint32(total) * uint32(4);
        end
        % 基址更新阶段不需要访问内存，mem_addr 保持默认值不影响



% ---- LDRD 链 ----
    case S_LDRD_R1
        mem_re   = true;
        mem_addr = uint32(addr);
        rdata_cap = uint32(mem_rdata);   % ★锁存第 1 字 [addr]

    case S_LDRD_WB1
        rf_we    = true;
        rf_addr  = uint8(ldrd_rt);
        rf_wdata = uint32(mem_rdata);   % 输入此时=读1数据，直接用
        mem_re   = true;
        mem_addr = uint32(addr) + uint32(4);

    case S_LDRD_R2
        rdata_cap = uint32(mem_rdata);  % 输入此时=读2数据，锁存

    case S_LDRD_WB2
        rf_we    = true;
        rf_addr  = uint8(ldrd_rt2);
        rf_wdata = rdata_cap;

    otherwise
        % S_IDLE / S_SCAN：默认值
end
end

== matlab function Three_Stages/ALU/MATLAB Function1 ==
  data: alu_a input; alu_v output; alu_b input; alu_result input; alu_op input
function alu_v = flags_v(alu_a, alu_b, alu_result, alu_op)
% =========================================================
% 计算 ALU 的 V (溢出) 标志
% 输入: alu_a, alu_b, alu_result, alu_op
% 输出: alu_v (boolean)
% =========================================================

    % ---------- 常量 ----------
    ALU_ADD = uint8(0);
    ALU_SUB = uint8(1);
    ALU_ADC = uint8(2);
    ALU_SBC = uint8(3);
    ALU_RSB = uint8(4);

    % ---------- 默认值 ----------
    alu_v = false;

    % ---------- 提取符号位 ----------
    a31 = logical(bitget(alu_a, 32));
    b31 = logical(bitget(alu_b, 32));
    r31 = logical(bitget(alu_result, 32));

    % ---------- 主逻辑 ----------
    if alu_op == ALU_ADD || alu_op == ALU_ADC
        % 加法溢出: 同号相加，结果变号
        alu_v = (a31 == b31) && (r31 ~= a31);

    elseif alu_op == ALU_SUB || alu_op == ALU_SBC
        % 减法溢出: 异号相减，结果变号 (结果与 a 不同号)
        alu_v = (a31 ~= b31) && (r31 ~= a31);

    elseif alu_op == ALU_RSB
        % RSB: b - a 的溢出
        alu_v = (b31 ~= a31) && (r31 ~= b31);

    else
        % 其他运算: V 恒为 0
        alu_v = false;
    end
end

== matlab function Three_Stages/ALU/MATLAB Function ==
  data: alu_a input; alu_c output; alu_b input; alu_result input; alu_op input; alu_carry_in input
function alu_c = flags_c(alu_a, alu_b, alu_result, alu_op, alu_carry_in)
% =========================================================
% 计算 ALU 的 C (进位/无借位) 标志
% 与更新后的 ALU.v 一致
% =========================================================

    % ---------- 常量 ----------
    ALU_ADD = uint8(0);
    ALU_SUB = uint8(1);
    ALU_ADC = uint8(2);
    ALU_SBC = uint8(3);
    ALU_RSB = uint8(4);

    % ---------- 默认值 ----------
    alu_c = false;

    % ---------- 用 uint64 做 33 位扩展加法 ----------
    a64 = uint64(alu_a);
    b64 = uint64(alu_b);
    c64 = uint64(alu_carry_in);      % boolean → uint64 (0 或 1)
    TWO32 = uint64(4294967296);      % 2^32

    % ---------- 主逻辑 ----------
    if alu_op == ALU_ADD
        % C = add_ext[32]，等价于 (a + b) >= 2^32
        sum64 = a64 + b64;
        alu_c = (sum64 >= TWO32);

    elseif alu_op == ALU_ADC
        % C = (a + b + carry_in) >= 2^32
        sum64 = a64 + b64 + c64;
        alu_c = (sum64 >= TWO32);

    elseif alu_op == ALU_SUB
        % C = ~borrow = (a >= b)
        alu_c = (a64 >= b64);

    elseif alu_op == ALU_SBC
        % a - b - ~carry_in  =>  无借位时 C=1
        % ~carry_in: carry_in=1 时为 0；carry_in=0 时为 1
        if alu_carry_in
            alu_c = (a64 >= b64);
        else
            alu_c = (a64 >= b64 + uint64(1));
        end

    elseif alu_op == ALU_RSB
        % C = (b >= a)
        alu_c = (b64 >= a64);

    else
        % 其他运算 C = 0
        alu_c = false;
    end
end
